simulink model "spring_mass_damper"  (R2025b)
settings: Solver=VariableStepAuto  StartTime=0.0  StopTime=30  MaxStep=0.001  RelTol=1e-3
settings Model: Creator=Shriram  LastModifiedBy=Shriram

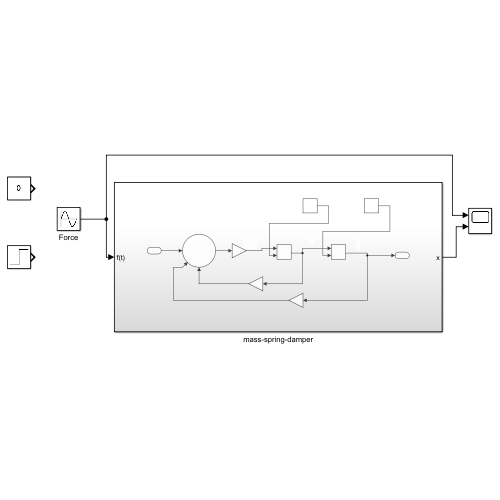
[thumbnail: Simulink's stored preview of the top-level diagram]
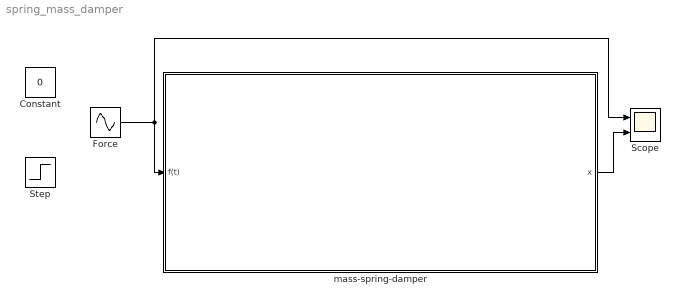
== system spring_mass_damper ==
  Constant : Constant  Value=0
  Force : Sin  Amplitude=2  Frequency=2  SampleTime=0
  Scope : Scope  NumInputPorts=2
      settings: ActiveDisplayYMinimum=-2.4999999965425634  ActiveDisplayYMaximum=2.4999999992410507
  Step : Step  SampleTime=0
  mass-spring-damper : Subsystem
  wires:
  Force/1 -> mass-spring-damper/1(f(t)), Scope/1
  mass-spring-damper/1(x) -> Scope/2

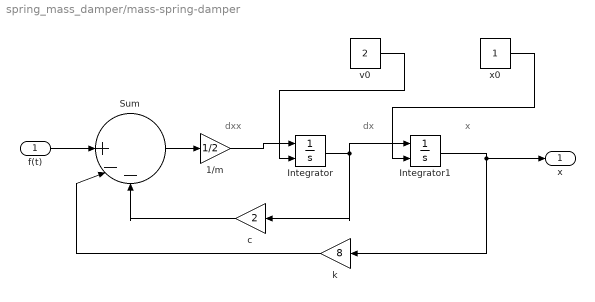
== system spring_mass_damper/mass-spring-damper ==
  note: x
  note: dx
  note: dxx
  f(t) : Inport
  1/m : Gain  Gain=1/2
  Integrator : Integrator  InitialConditionSource=external  InitialCondition=2
  Integrator1 : Integrator  InitialConditionSource=external  InitialCondition=1
  Sum : Sum  Inputs=||+--
  c : Gain  Gain=2
  k : Gain  Gain=8
  v0 : Constant  Value=2
  x0 : Constant
  x : Outport
  wires:
  Integrator1/1 -> x/1, k/1
  c/1 -> Sum/3
  Integrator/1 -> Integrator1/1, c/1
  k/1 -> Sum/2
  Sum/1 -> 1/m/1
  1/m/1 -> Integrator/1
  f(t)/1 -> Sum/1
  v0/1 -> Integrator/2
  x0/1 -> Integrator1/2
